simulink library "snake_single_module_library_torque_multi"  (R2025a)
settings: Solver=VariableStepAuto  StartTime=0.0  StopTime=10.0  RelTol=1e-3
values from neighbouring files (symbols this model uses):
  N = 29    [Stiffness_cal.m]    (also in m20260427_3_testing_config2torque.m = 1; m20260831_1_testing_config2torque.m; process_two_imus.m = size(q1_xyzw,1); run_compye_theta_phi_from_file.m = size(RRel, 3))
libraries: snake_subsystem_torque x29, sm_lib x2
settings Model: Creator=dperera  LastModifiedBy=dperera

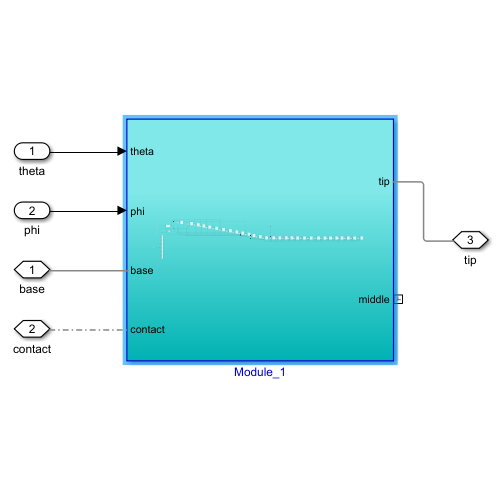
[thumbnail: Simulink's stored preview of the top-level diagram]
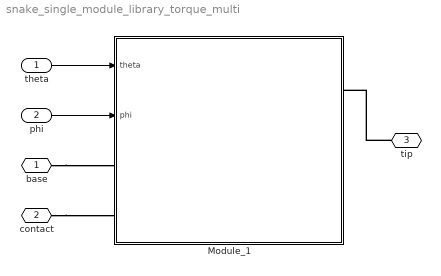
== system snake_single_module_library_torque_multi ==
  theta : Inport
  phi : Inport  Port=2
  Module_1 : Subsystem
  base : PMIOPort  Side=Left
  contact : PMIOPort  Port=2  Side=Left
  tip : PMIOPort  Port=3  Side=Right
  wires:
  theta/1 -> Module_1/1(theta)
  phi/1 -> Module_1/2(phi)
  connections:
  base/RConn1 -- Module_1/LConn1
  tip/RConn1 -- Module_1/RConn1
  contact/RConn1 -- Module_1/LConn2

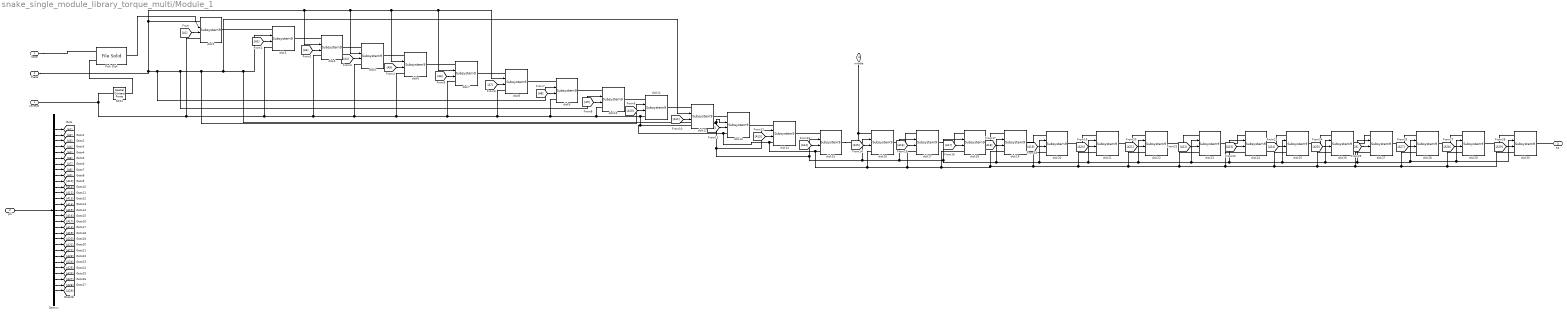
== system snake_single_module_library_torque_multi/Module_1 ==
  theta : Inport
  phi : Inport  Port=2
  " Pink Disk" : sm_lib/Body Elements/File Solid  ExtGeomFileName=\Snake_Locomotion_Solidworks\SL_Disk.STEP  UnitType=FromFile  ExtGeomFileUnits=m  StepReaderType=HEX  ExportConvexHullGeometry=on  InertiaType=CalculateFromGeometry  BasedOnType=Mass  Density=1000  DensityUnits=kg/m^3  Mass=100/30  MassUnits=g  CenterOfMass=[0 0 0]  CenterOfMassUnits=m  MomentsOfInertia=[1 1 1]  MomentsOfInertiaUnits=kg*m^2  ProductsOfInertia=[0 0 0]  ProductsOfInertiaUnits=kg*m^2  GraphicType=FromGeometry  MarkerShape=Frame  MarkerSize=1000  GraphicVisPropType=SimpleVisualProperties  GraphicDiffuseColor=[1 0 0]  GraphicOpacity=1  GraphicSpecularColor=[0.5 0.5 0.5 1.0]  GraphicAmbientColor=[0.15 0.15 0.15 1.0]  GraphicEmissiveColor=[0.0 0.0 0.0 1.0]  GraphicShininess=75  DoExposeReferenceFrame=off  SerializedFrames=<Frames><Frame><Id>Frame1</Id><Value><Name>Center</Name><Origin><Source>ReferenceFrame</Source><FeatureName></FeatureName></Origin><PrimaryAxis><DefinedDirection>+Z</DefinedDirection><Source>ReferenceFrame</Source><SourceDirection>+Z</SourceDirection><FeatureName></FeatureName></PrimaryAxis><SecondaryAxis><DefinedDirection>+X</DefinedDirection><Source>ReferenceFrame</Source><SourceDirection>+X</SourceDirection><FeatureName></FeatureName></SecondaryAxis></Value></Frame><Frame><Id>Frame2</Id><Value><Name>F2</Name><Origin><Source>ReferenceFrame</Source><FeatureName></FeatureName></Origin><PrimaryAxis><DefinedDirection>+Z</DefinedDirection><Source>ReferenceFrame</Source><SourceDirection>+Z</SourceDirection><FeatureName></FeatureName></PrimaryAxis><SecondaryAxis><DefinedDirection>+X</DefinedDirection><Source>ReferenceFrame</Source><SourceDirection>+X</SourceDirection><FeatureName></FeatureName></SecondaryAxis></Value></Frame></Frames>
  Demux : Demux  Outputs=29
  SCF1 : sm_lib/Forces and Torques/Spatial Contact Force  SenseSeparationDistance=off  NormalForceType=SmoothSpringDamper  NormalStiffness=1e8  NormalStiffnessUnits=N/m  NormalDamping=1e3  NormalDampingUnits=N/(m/s)  NormalTransitionRegionWidth=1e-4  NormalTransitionRegionWidthUnits=m  FrictionType=SmoothStickSlip  CoefficientOfStaticFriction=5  CoefficientOfDynamicFriction=2  FrictionalCriticalVelocity=0.1  FrictionalCriticalVelocityUnits=m/s  SenseContactSignal=off  SensePenetrationDepth=off  SenseNormalVelocity=off  SenseTangentialVelocity=off  SensingForceTorqueDirection=BaseOnFollower  SensingForceTorqueResolutionFrame=ContactFrame  SenseNormalForce=off  SenseNormalForceMagnitude=off  SenseNormalTorque=off  SenseFrictionalForce=off  SenseFrictionalForceMagnitude=off  SenseFrictionalTorque=off  SenseTotalForce=off  SenseTotalTorque=off  SenseContactBaseRotation=off  SenseContactBaseTranslation=off  SenseContactFollowerRotation=off  SenseContactFollowerTranslation=off  ZeroCrossDetectContactStartAndEnd=off
  disk{2..30} (29 alike) : snake_subsystem_torque/Subsystem9  SystemSampleTime=-1  VariantActivationTime=update diagram  EmptyChoice=off  PassThrough=off  PassThroughVariantControl=(default)  EmptyChoiceVariantControl=(default)  AllowFlexibleInterface=on  Latency=0  AutoFrameSizeCalculation=off
      settings: PortSchema="{\"entries\":[{\"content\":{\"sides\":[{\"content\":{\"connectorIds\":[\"LConn1\",\"In1\",\"In2\",\"LConn2\"]},\"type\":\"ConnectorPlacement.EquallySpacedRectSide\",\"uuid\":\"3bbd7745-fe2e-4e9d-a66d-a186a50d348a\"},{\"content\":{\"connectorIds\":[\"RConn1\"],\"side\":\"RIGHT\"},\"type\":\"ConnectorPlacement.EquallySpacedRectSide\",\"uuid\":\"c5ce652e-a2c8-4f5d-9e32-f3f4c638c96f\"},{\"content\":{\"side\":\"TOP\"},\"type\":\"ConnectorPlacement.EquallySpacedRectSide\",\"uuid\":\"058fc2a1-1a1b-48b6-a1cd-b102d1de0895\"}]},\"type\":\"ConnectorPlacement.EquallySpacedConnector\",\"uuid\":\"f4c16c24-b963-4a18-943c-17003bfc54e7\"}],\"packageUris\":[\"http://schema.mathworks.com/mf0/Connector/R2020b\"],\"version\":\"1.0\"}"
  base : PMIOPort  Side=Left
  contact : PMIOPort  Port=2  Side=Left
  tip : PMIOPort  Port=3  Side=Right
  middle : PMIOPort  Port=4  Side=Right
  wires:
  theta/1 -> disk2/1, disk4/1, disk5/1, disk6/1, disk8/1, disk7/1, disk9/1, disk10/1, disk11/1, disk12/1, disk3/1, disk13/1, disk14/1, disk15/1, disk16/1, disk17/1, disk18/1, disk19/1, disk20/1, disk21/1, disk22/1, disk23/1, disk24/1, disk25/1, disk26/1, disk27/1, disk28/1, disk29/1, disk30/1
  phi/1 -> Demux/1
  Demux/1 -> [A1]
  [A1] -> disk2/2
  Demux/2 -> [A2]
  [A2] -> disk3/2
  Demux/3 -> [A3]
  [A3] -> disk4/2
  Demux/4 -> [A4]
  [A4] -> disk5/2
  Demux/5 -> [A5]
  [A5] -> disk6/2
  Demux/6 -> [A6]
  [A6] -> disk7/2
  Demux/7 -> [A7]
  [A7] -> disk8/2
  Demux/8 -> [A8]
  [A8] -> disk9/2
  Demux/9 -> [A9]
  [A9] -> disk10/2
  Demux/10 -> [A10]
  [A10] -> disk11/2
  Demux/11 -> [A11]
  [A11] -> disk12/2
  Demux/12 -> [A12]
  [A12] -> disk13/2
  Demux/13 -> [A13]
  [A13] -> disk14/2
  Demux/14 -> [A14]
  [A14] -> disk15/2
  Demux/15 -> [A15]
  [A15] -> disk16/2
  Demux/16 -> [A16]
  [A16] -> disk17/2
  Demux/17 -> [A17]
  [A17] -> disk18/2
  Demux/18 -> [A18]
  [A18] -> disk19/2
  Demux/19 -> [A19]
  [A19] -> disk20/2
  Demux/20 -> [A20]
  [A20] -> disk21/2
  Demux/21 -> [A21]
  [A21] -> disk22/2
  Demux/22 -> [A22]
  [A22] -> disk23/2
  Demux/23 -> [A23]
  [A23] -> disk24/2
  Demux/24 -> [A24]
  [A24] -> disk25/2
  Demux/25 -> [A25]
  [A25] -> disk26/2
  Demux/26 -> [A26]
  [A26] -> disk27/2
  Demux/27 -> [A27]
  [A27] -> disk28/2
  Demux/28 -> [A28]
  [A28] -> disk29/2
  Demux/29 -> [A29]
  [A29] -> disk30/2
  connections:
  disk2/LConn1 -- " Pink Disk"/RConn1
  disk12/LConn1 -- disk11/RConn1
  disk3/LConn1 -- disk2/RConn1
  disk5/LConn1 -- disk4/RConn1
  disk11/LConn1 -- disk10/RConn1
  disk4/LConn1 -- disk3/RConn1
  " Pink Disk"/LConn2 -- SCF1/RConn1
  disk6/LConn1 -- disk5/RConn1
  disk14/LConn1 -- disk13/RConn1
  disk9/LConn1 -- disk8/RConn1
  disk13/LConn1 -- disk12/RConn1
  disk7/LConn1 -- disk6/RConn1
  disk8/LConn1 -- disk7/RConn1
  disk10/LConn1 -- disk9/RConn1
  base/RConn1 -- " Pink Disk"/LConn1
  disk15/LConn1 -- disk14/RConn1
  middle/RConn1 -- disk16/LConn1 -- disk15/RConn1
  disk17/LConn1 -- disk16/RConn1
  disk17/RConn1 -- disk18/LConn1
  disk18/RConn1 -- disk19/LConn1
  disk20/LConn1 -- disk19/RConn1
  disk21/LConn1 -- disk20/RConn1
  disk22/LConn1 -- disk21/RConn1
  disk23/LConn1 -- disk22/RConn1
  disk24/LConn1 -- disk23/RConn1
  disk25/LConn1 -- disk24/RConn1
  disk26/LConn1 -- disk25/RConn1
  disk27/LConn1 -- disk26/RConn1
  disk28/LConn1 -- disk27/RConn1
  disk29/LConn1 -- disk28/RConn1
  disk30/LConn1 -- disk29/RConn1
  disk3/LConn2 -- disk2/LConn2 -- SCF1/LConn1 -- contact/RConn1 -- disk4/LConn2 -- disk5/LConn2 -- disk6/LConn2 -- disk7/LConn2 -- disk8/LConn2 -- disk9/LConn2 -- disk12/LConn2 -- disk30/LConn2 -- disk29/LConn2 -- disk28/LConn2 -- disk27/LConn2 -- disk26/LConn2 -- disk25/LConn2 -- disk24/LConn2 -- disk23/LConn2 -- disk22/LConn2 -- disk21/LConn2 -- disk20/LConn2 -- disk19/LConn2 -- disk18/LConn2 -- disk17/LConn2 -- disk16/LConn2 -- disk15/LConn2 -- disk14/LConn2 -- disk13/LConn2 -- disk11/LConn2 -- disk10/LConn2
  tip/RConn1 -- disk30/RConn1
